simulink model "sst_cllc_dcx_35kHz"  (R2026b)
settings: Solver=ode23tb  StopTime=param.sim.simlength  FixedStep=tc  MaxStep=param.glb_time.tc
values from neighbouring files (symbols this model uses):
  param = struct()    [init_model.m]
libraries: fl_lib x144, nesl_utility x71, mos_simple_2th_lib x8, discrete_time_low_pass_filter x2, lithium_ion_battery x1, single_phase_transformer x1, dab_single_phase_pwm_modulator x1, ee_lib x1
(part 1 of 4)
settings Model: Creator=LTNBDA  LastModifiedBy=d.bagnara
settings SolverCC: AutoInsertRateTranBlk=on  SolverResetMethod=Robust  ZeroCrossAlgorithm=Adaptive  ZeroCrossControl=EnableAll
settings DataIOCC: DSMLogging=off  LimitDataPoints=on  MaxDataPoints=1  ReturnWorkspaceOutputs=off  SaveFormat=Array  SaveOutput=off  SaveTime=off  SignalLogging=off  SignalLoggingSaveFormat=ModelDataLogs
settings OptimizationCC: EfficientMapNaN2IntZero=off  LifeSpan=inf  MemsetInitFltsAndDblsToZero=off
settings DebuggingCC: ArithmeticOperatorsInVariantConditions=warning  FcnCallInpInsideContextMsg=warning  MergeDetectMultiDrivingBlocksExec=none  MultiTaskCondExecSysMsg=none  MultiTaskDSMMsg=warning  MultiTaskRateTransMsg=warning  SFNoUnconditionalDefaultTransitionDiag=warning  SFUnexpectedBacktrackingDiag=warning  SaveWithParameterizedLinksMsg=none  SignalResolutionControl=TryResolveAllWithWarning  SolverPrmCheckMsg=warning  StateNameClashWarn=warning
settings HardwareCC: ProdEndianess=Unspecified  ProdEqTarget=off  ProdHWDeviceType=Generic->64-bit Embedded Processor (LP64)  ProdIntDivRoundTo=Undefined  ProdLargestAtomicFloat=None  TargetEndianess=LittleEndian  TargetHWDeviceType=MATLAB Host  TargetIntDivRoundTo=Zero  TargetLongLongMode=on
settings ModelReferenceCC: PropagateSignalLabelsOutOfModel=off
settings SFSimCC: CustomCodeUndefinedFunction=UseInterfaceOnly  SimUseLocalCustomCode=off
settings SFSimCC: SimCustomHeaderCode=|
  | #include "rpi.h"
  | #include "rpi_simulink.h"
  | #include "mavgflt.h"
  | #include "mavgflt_simulink.h"
  | #include "bemf_obsv.h"
  | #include "bemf_obsv_simulink.h"
  | #include "bemf_obsv_load_est.h"
  | #include "bemf_obsv_load_est_simulink.h"
  | #include "dqvector_pi.h"
  | #include "dqvector_pi_simulink.h"
  | #include "sv_pwm_simulink.h"
  | #include "sv_pwm.h"
  | #include "first_harmonic_tracker.h"
  | #include "first_harmonic_tracker_simulink.h"
  | #include "dqpll_thyr.h"
  | #include "dqpll_thyr_simulink.h"
  | #include "dqpll_grid.h"
  | #include "dqpll_grid_simulink.h"
settings SFSimCC: SimUserIncludeDirs=|
  | include
  | src
settings SFSimCC: SimUserSources=|
  | "mavgflt_simulink.c"
  | "mavgflt.c"
  | "bemf_obsv_simulink.c"
  | "bemf_obsv.c"
  | "bemf_obsv_load_est_simulink.c"
  | "bemf_obsv_load_est.c"
  | "dqvector_pi.c"
  | "dqvector_pi_simulink.c"
  | "sv_pwm_simulink.c"
  | "sv_pwm.c"
  | "first_harmonic_tracker_simulink.c"
  | "first_harmonic_tracker.c"
  | "dqpll_thyr_simulink.c"
  | "dqpll_thyr.c"
  | "dqpll_grid_simulink.c"
  | "dqpll_grid.c"
  | "rpi_simulink.c"
  | "rpi.c"
settings RTWCC: RTWUseLocalCustomCode=off
settings CodeAppCC: StateflowObjectComments=on
settings GRTTargetCC: CombineOutputUpdateFcns=off  GRTInterface=on  TargetLangStandard=C89/C90 (ANSI)
settings ConfigComp: CovExternalEMLEnable=off  CovSaveCumulativeToWorkspaceVar=on  CovSaveSingleToWorkspaceVar=on
settings SimscapeCC: SimscapeNormalizeSystem=off  SimscapeUseEnergyAccounting=off

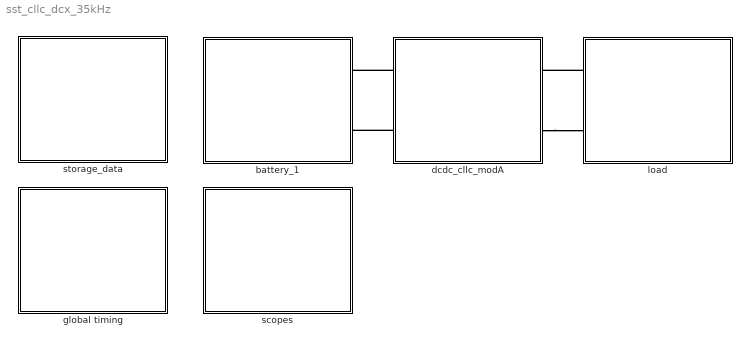
== system sst_cllc_dcx_35kHz ==
  battery_1 : Subsystem
  dcdc_cllc_modA : Subsystem
  global timing : Subsystem
  load : Subsystem
  scopes : Subsystem
  storage_data : Subsystem
  connections:
  dcdc_cllc_modA/LConn1 -- battery_1/RConn1
  dcdc_cllc_modA/LConn2 -- battery_1/RConn2
  load/LConn1 -- dcdc_cllc_modA/RConn1
  dcdc_cllc_modA/RConn2 -- load/LConn2

== system sst_cllc_dcx_35kHz/battery_1 ==
  Electrical Reference1 : fl_lib/Electrical/Electrical Elements/Electrical Reference
  Resistor : fl_lib/Electrical/Electrical Elements/Resistor  Commented=on  R=param.cllc.sink.R1 Ohm  i_specify=off  i_priority=None  i=0 A  i_nominal_specify=off  i_nominal_value=1  i_nominal_unit=A  v_specify=off  v_priority=None  v=0 V  v_nominal_specify=off  v_nominal_value=1  v_nominal_unit=V
  Solver Configuration : nesl_utility/Solver Configuration  PhysicalDomain=network_engine_domain  SubClassName=solver  LeftPortType=input  RightPortType=generic  Tones=[]  Harmonics=[]  SimulateNoise=off  Profile=off  UseLocalSampling=off  EnableSwitchedLinearOptims=on  FrequencyDomain=off  UseCCode=off  RelTol=0.001  AbsTol=0.001  MinStep=1e-09  ToWorkspace=off  RevertToSquareIcSolve=off  NumHomotopyIterations=100  PhasorMode=off  PhasorModeNumHarmonics=1  ConsistencySolver=NEWTON_FTOL  CanonicalOrdering=UNORDERED  OptimizeIntermediates=UNOPTIMIZED  MulticoreSolverChoice=BACKWARD_EULER  IndexReductionMethod=DerivativeReplacement  DoDC=on  ResidualTolerance=1e-5  ConsistencyTolSource=GLOBAL  ConsistencyAbsTol=0.001  ConsistencyRelTol=0.001  ConsistencyTolFactor=0.001  UseLocalSolver=on  LocalSolverChoice=NE_BACKWARD_EULER_ADVANCER  ResolveIndetEquations=on  FunctionEvalNumThread=1  LocalSolverSampleTime=param.glb_time.tc  DoFixedCost=on  MaxNonlinIter=param.sim.nonlinear_iterations  MaxModeIter=2  ComputeImpulses=off  ImpulseIterations=2  LinearAlgebra=auto  LinearAlgebraNumThread=0  EquationFormulation=NE_TIME_EF  DelaysMemoryBudget=1024  AutomaticFiltering=on  FilteringTimeConstant=0.001  PartitionStorageMethod=AS_NEEDED  PartitionMemoryBudget=1024  PartitionMethod=BALANCED  MultibodyUseLocalSolver=off  MultibodyLocalSolverChoice=ODE1  MultibodyLocalSolverSampleTime=0.001
  To Workspace14 : ToWorkspace  VariableName=battery_1_data_sim  SampleTime=param.glb_time.tc
      settings: MaxDataPoints=param.glb_time.Nc  Decimation=param.glb_time.decimation_tc
  lithium ion battery : Scope
      settings: ActiveDisplayYMinimum=-190.26234523392469  ActiveDisplayYMaximum=789.35449820003043  DataLoggingVariableName=ScopeData3
  lithium_ion_battery : lithium_ion_battery/lithium_ion_battery  Q=param.battery.pack_1.Q  number_of_cells=param.battery.pack_1.number_of_cells  E_1=param.battery.pack_1.E_1  E0=param.battery.pack_1.E0  E1=param.battery.pack_1.E1  E2=param.battery.pack_1.E2  E3=param.battery.pack_1.E3  Elog=param.battery.pack_1.Elog  R0=param.battery.pack_1.R0  R1=param.battery.pack_1.R1  C1=param.battery.pack_1.C1  M=param.battery.pack_1.M  alpha=param.battery.pack_1.alpha  soc_init=param.battery.pack_1.soc_init  ts_battery=param.glb_time.ts_dab  q1Kalman=param.battery.pack_1.q1Kalman  q2Kalman=param.battery.pack_1.q2Kalman  q3Kalman=param.battery.pack_1.q3Kalman  rKalman=param.battery.pack_1.rKalman  tc=param.glb_time.tc  enable_white_noise_m=1  battery_voltage_init_m=param.battery.nominal_battery_voltage_1
  single_phase_ui_measure : Subsystem
  dc(+) : PMIOPort  Side=Right
  dc(-) : PMIOPort  Port=2  Side=Right
  wires:
  lithium_ion_battery/1 -> To Workspace14/1, lithium ion battery/1
  connections:
  lithium_ion_battery/RConn2 -- Resistor/RConn1 -- single_phase_ui_measure/LConn2 -- Electrical Reference1/LConn1 -- Solver Configuration/RConn1
  single_phase_ui_measure/RConn1 -- dc(+)/RConn1
  single_phase_ui_measure/LConn1 -- Resistor/LConn1 -- lithium_ion_battery/RConn1
  dc(-)/RConn1 -- single_phase_ui_measure/RConn2

== system sst_cllc_dcx_35kHz/dcdc_cllc_modA ==
  dc/dc with galvanic isolation : Subsystem
  input_current_control : Subsystem
  udc(+) : PMIOPort  Side=Right
  udc(-) : PMIOPort  Port=2  Side=Right
  dc(+) : PMIOPort  Port=3  Side=Left
  dc(-) : PMIOPort  Port=4  Side=Left
  wires:
  input_current_control/1(gate_cmds) -> dc/dc with galvanic isolation/1(dab_gate_cmds)
  connections:
  udc(+)/RConn1 -- dc/dc with galvanic isolation/RConn1
  udc(-)/RConn1 -- dc/dc with galvanic isolation/RConn2
  dc(-)/RConn1 -- dc/dc with galvanic isolation/LConn2
  dc(+)/RConn1 -- dc/dc with galvanic isolation/LConn1

== system sst_cllc_dcx_35kHz/global timing ==
  Unit Delay : UnitDelay  SampleTime=param.glb_time.tc
  time_afe1 : Subsystem  mask{k=1}
      mask prompts: k "Time Gain"
      mask Display:
      | disp('time-gen');
      | port_label('input', 1, 'crt');
      | port_label('output', 1, 'tout');
  time_afe3 : Subsystem  mask{k=1}
      mask prompts: k "Time Gain"
      mask Display:
      | disp('time-gen');
      | port_label('output', 1, 'tout');
  tag scope: time_cllc_module_1=global, time_master=global
  wires:
  time_afe1/1(Out1) -> [time_cllc_module_1]
  time_afe3/1(Out1) -> [time_master]
  [local_time_corr_llc_mod1] -> Unit Delay/1
  Unit Delay/1 -> time_afe1/1(correction_time)

== system sst_cllc_dcx_35kHz/load ==
  Clock : Clock  Commented=on
  Controlled Current Source : fl_lib/Electrical/Electrical Sources/Controlled Current Source  Commented=on
  Electrical Reference1 : fl_lib/Electrical/Electrical Elements/Electrical Reference
  Gain : Gain  Commented=on  Gain=1/param.cllc.sink.t_ramp
  Gain1 : Gain  Commented=on  Gain=param.cllc.sink.I2
  Saturation : Saturate  Commented=on  UpperLimit=1  LowerLimit=0
  Simulink-PS Converter : nesl_utility/Simulink-PS Converter  Commented=on  PhysicalDomain=network_engine_domain  SubClassName=ps_input  LeftPortType=input  RightPortType=output  PseudoPeriodic=off  Frequencies=[]  NoiseDistribution=none  NoiseParameters=[]  Unit=A  AffineConversion=off  FilteringAndDerivatives=provide  SimscapeFilterOrder=1  InputFilterTimeConstant=0.001  UdotUserProvided=0
  Voltage Source : ee_lib/Sources/Voltage Source  Commented=on  dc_voltage=param.cllc.sink.U2 V  ac_voltage=0 V  ac_shift=0 rad  ac_frequency=0 Hz  noise_mode=ee.enum.sources.noise.Disabled  PSD=0 V^2/Hz  sample_time=1e-3 s  repeatability=ee.enum.sources.repeatability.NotRepeatable  user_seed=0  auto_seed=3499211588  i_specify=off  i_priority=None  i=0 A  i_nominal_specify=off  i_nominal_value=1  i_nominal_unit=A  v_specify=off  v_priority=None  v=0 V  v_nominal_specify=off  v_nominal_value=1  v_nominal_unit=V
  passive load : Subsystem
  uload(+) : PMIOPort  Side=Left
  uload(-) : PMIOPort  Port=2  Side=Left
  wires:
  Clock/1 -> Gain/1
  Gain/1 -> Saturation/1
  Saturation/1 -> Gain1/1
  Gain1/1 -> Simulink-PS Converter/1
  connections:
  uload(-)/RConn1 -- Controlled Current Source/LConn1 -- Voltage Source/RConn1 -- Electrical Reference1/LConn1 -- passive load/RConn1
  passive load/LConn1 -- Controlled Current Source/RConn2 -- Voltage Source/LConn1 -- uload(+)/RConn1
  Simulink-PS Converter/RConn1 -- Controlled Current Source/RConn1

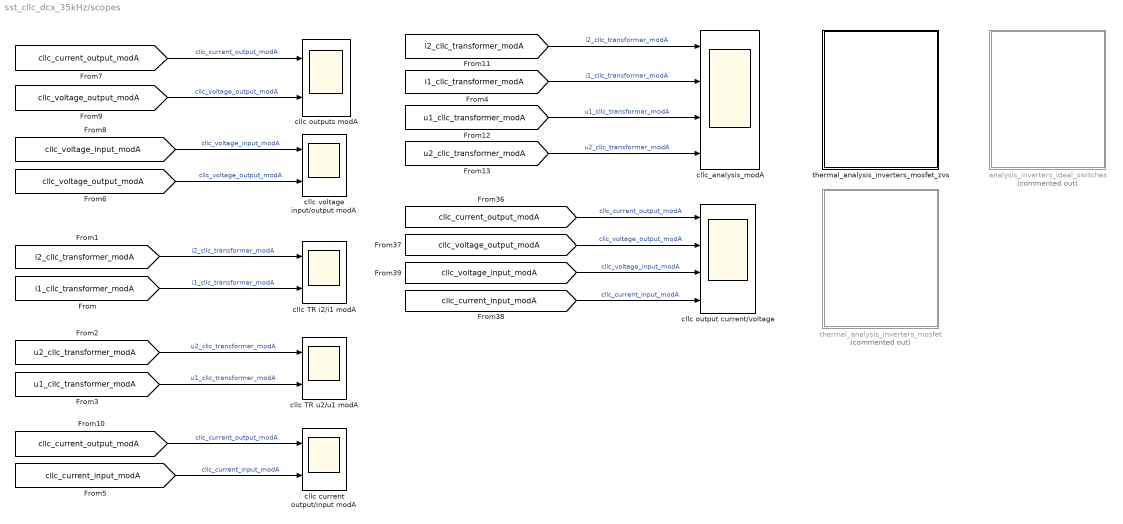
== system sst_cllc_dcx_35kHz/scopes ==
  analysis_inverters_ideal_switches : Subsystem  Commented=on
  cllc TR i2/i1 modA : Scope  NumInputPorts=2
      settings: SampleTime=param.glb_time.tc  ActiveDisplayYMinimum=-621.44843192916471  ActiveDisplayYMaximum=621.071538249071  DataLoggingVariableName=ScopeData13
  cllc TR u2/u1 modA : Scope  NumInputPorts=2
      settings: SampleTime=param.glb_time.tc  ActiveDisplayYMinimum=-1427.1389570347349  ActiveDisplayYMaximum=1427.1405694303187  DataLoggingVariableName=ScopeData4
  cllc current output/input modA : Scope  NumInputPorts=2
      settings: SampleTime=param.glb_time.tc  ActiveDisplayYMinimum=-7.8124999999999982  ActiveDisplayYMaximum=70.3125  DataLoggingVariableName=ScopeData8
  cllc output current/voltage : Scope  NumInputPorts=4
      settings: ActiveDisplayString=3  ActiveDisplayYMinimum=656.54883928896152  ActiveDisplayYMaximum=674.48308776467979  DataLoggingVariableName=ScopeData9
  cllc outputs modA : Scope  NumInputPorts=2
      settings: ActiveDisplayYMinimum=791.98525003287466  ActiveDisplayYMaximum=792.09422024718685  DataLoggingVariableName=ScopeData6
  cllc voltage input/output modA : Scope  NumInputPorts=2
      settings: ActiveDisplayYMinimum=778.88698009854056  ActiveDisplayYMaximum=810.81441530748316  DataLoggingVariableName=ScopeData10
  cllc_analysis_modA : Scope  NumInputPorts=4
      settings: ActiveDisplayYMinimum=-2946.4603447985373  ActiveDisplayYMaximum=3872.2014328676551  DataLoggingVariableName=ScopeData15
  thermal_analysis_inverters_mosfet : Subsystem  Commented=on
  thermal_analysis_inverters_mosfet_zvs : Subsystem
  wires:
  [u2_cllc_transformer_modA] -> cllc TR u2/u1 modA/1  "u2_cllc_transformer_modA"
  [i1_cllc_transformer_modA] -> cllc_analysis_modA/2  "i1_cllc_transformer_modA"
  [cllc_current_output_modA] -> cllc current output/input modA/1  "cllc_current_output_modA"
  [cllc_current_input_modA] -> cllc current output/input modA/2  "cllc_current_input_modA"
  [cllc_voltage_output_modA] -> cllc outputs modA/2  "cllc_voltage_output_modA"
  [cllc_current_output_modA] -> cllc outputs modA/1  "cllc_current_output_modA"
  [i2_cllc_transformer_modA] -> cllc_analysis_modA/1  "i2_cllc_transformer_modA"
  [cllc_voltage_output_modA] -> cllc output current/voltage/2  "cllc_voltage_output_modA"
  [u1_cllc_transformer_modA] -> cllc_analysis_modA/3  "u1_cllc_transformer_modA"
  [cllc_voltage_output_modA] -> cllc voltage input/output modA/2  "cllc_voltage_output_modA"
  [i1_cllc_transformer_modA] -> cllc TR i2/i1 modA/2  "i1_cllc_transformer_modA"
  [cllc_current_input_modA] -> cllc output current/voltage/4  "cllc_current_input_modA"
  [i2_cllc_transformer_modA] -> cllc TR i2/i1 modA/1  "i2_cllc_transformer_modA"
  [cllc_voltage_input_modA] -> cllc voltage input/output modA/1  "cllc_voltage_input_modA"
  [u1_cllc_transformer_modA] -> cllc TR u2/u1 modA/2  "u1_cllc_transformer_modA"
  [u2_cllc_transformer_modA] -> cllc_analysis_modA/4  "u2_cllc_transformer_modA"
  [cllc_voltage_input_modA] -> cllc output current/voltage/3  "cllc_voltage_input_modA"
  [cllc_current_output_modA] -> cllc output current/voltage/1  "cllc_current_output_modA"

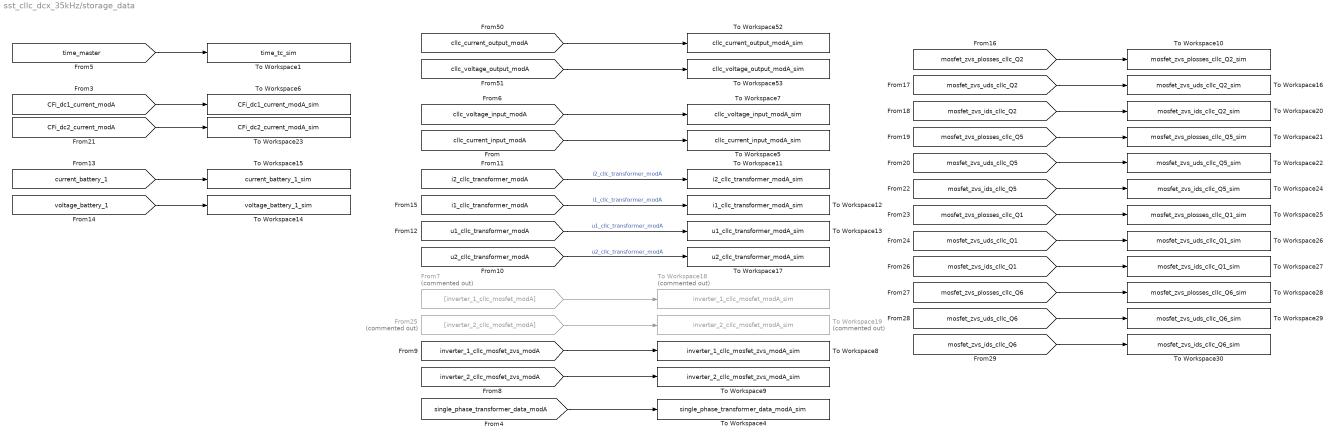
== system sst_cllc_dcx_35kHz/storage_data ==
  From25 : From  Commented=on  GotoTag=inverter_2_cllc_mosfet_modA
  From7 : From  Commented=on  GotoTag=inverter_1_cllc_mosfet_modA
  To Workspace1 : ToWorkspace  VariableName=time_tc_sim  SampleTime=param.glb_time.tc
      settings: MaxDataPoints=param.glb_time.Nc  Decimation=param.glb_time.decimation_tc
  To Workspace10 : ToWorkspace  VariableName=mosfet_zvs_plosses_cllc_Q2_sim  SampleTime=param.glb_time.tc
      settings: MaxDataPoints=param.glb_time.Nc  Decimation=param.glb_time.decimation_tc
  To Workspace11 : ToWorkspace  VariableName=i2_cllc_transformer_modA_sim  SampleTime=param.glb_time.tc
      settings: MaxDataPoints=param.glb_time.Nc  Decimation=param.glb_time.decimation_tc
  To Workspace12 : ToWorkspace  VariableName=i1_cllc_transformer_modA_sim  SampleTime=param.glb_time.tc
      settings: MaxDataPoints=param.glb_time.Nc  Decimation=param.glb_time.decimation_tc
  To Workspace13 : ToWorkspace  VariableName=u1_cllc_transformer_modA_sim  SampleTime=param.glb_time.tc
      settings: MaxDataPoints=param.glb_time.Nc  Decimation=param.glb_time.decimation_tc
  To Workspace14 : ToWorkspace  VariableName=voltage_battery_1_sim  SampleTime=param.glb_time.tc
      settings: MaxDataPoints=param.glb_time.Nc  Decimation=param.glb_time.decimation_tc
  To Workspace15 : ToWorkspace  VariableName=current_battery_1_sim  SampleTime=param.glb_time.tc
      settings: MaxDataPoints=param.glb_time.Nc  Decimation=param.glb_time.decimation_tc
  To Workspace16 : ToWorkspace  VariableName=mosfet_zvs_uds_cllc_Q2_sim  SampleTime=param.glb_time.tc
      settings: MaxDataPoints=param.glb_time.Nc  Decimation=param.glb_time.decimation_tc
  To Workspace17 : ToWorkspace  VariableName=u2_cllc_transformer_modA_sim  SampleTime=param.glb_time.tc
      settings: MaxDataPoints=param.glb_time.Nc  Decimation=param.glb_time.decimation_tc
  To Workspace18 : ToWorkspace  Commented=on  VariableName=inverter_1_cllc_mosfet_modA_sim  SampleTime=param.glb_time.tc
      settings: MaxDataPoints=param.glb_time.Nc  Decimation=param.glb_time.decimation_tc
  To Workspace19 : ToWorkspace  Commented=on  VariableName=inverter_2_cllc_mosfet_modA_sim  SampleTime=param.glb_time.tc
      settings: MaxDataPoints=param.glb_time.Nc  Decimation=param.glb_time.decimation_tc
  To Workspace20 : ToWorkspace  VariableName=mosfet_zvs_ids_cllc_Q2_sim  SampleTime=param.glb_time.tc
      settings: MaxDataPoints=param.glb_time.Nc  Decimation=param.glb_time.decimation_tc
  To Workspace21 : ToWorkspace  VariableName=mosfet_zvs_plosses_cllc_Q5_sim  SampleTime=param.glb_time.tc
      settings: MaxDataPoints=param.glb_time.Nc  Decimation=param.glb_time.decimation_tc
  To Workspace22 : ToWorkspace  VariableName=mosfet_zvs_uds_cllc_Q5_sim  SampleTime=param.glb_time.tc
      settings: MaxDataPoints=param.glb_time.Nc  Decimation=param.glb_time.decimation_tc
  To Workspace23 : ToWorkspace  VariableName=CFi_dc2_current_modA_sim  SampleTime=param.glb_time.tc
      settings: MaxDataPoints=param.glb_time.Nc  Decimation=param.glb_time.decimation_tc
  To Workspace24 : ToWorkspace  VariableName=mosfet_zvs_ids_cllc_Q5_sim  SampleTime=param.glb_time.tc
      settings: MaxDataPoints=param.glb_time.Nc  Decimation=param.glb_time.decimation_tc
  To Workspace25 : ToWorkspace  VariableName=mosfet_zvs_plosses_cllc_Q1_sim  SampleTime=param.glb_time.tc
      settings: MaxDataPoints=param.glb_time.Nc  Decimation=param.glb_time.decimation_tc
  To Workspace26 : ToWorkspace  VariableName=mosfet_zvs_uds_cllc_Q1_sim  SampleTime=param.glb_time.tc
      settings: MaxDataPoints=param.glb_time.Nc  Decimation=param.glb_time.decimation_tc
  To Workspace27 : ToWorkspace  VariableName=mosfet_zvs_ids_cllc_Q1_sim  SampleTime=param.glb_time.tc
      settings: MaxDataPoints=param.glb_time.Nc  Decimation=param.glb_time.decimation_tc
  To Workspace28 : ToWorkspace  VariableName=mosfet_zvs_plosses_cllc_Q6_sim  SampleTime=param.glb_time.tc
      settings: MaxDataPoints=param.glb_time.Nc  Decimation=param.glb_time.decimation_tc
  To Workspace29 : ToWorkspace  VariableName=mosfet_zvs_uds_cllc_Q6_sim  SampleTime=param.glb_time.tc
      settings: MaxDataPoints=param.glb_time.Nc  Decimation=param.glb_time.decimation_tc
  To Workspace30 : ToWorkspace  VariableName=mosfet_zvs_ids_cllc_Q6_sim  SampleTime=param.glb_time.tc
      settings: MaxDataPoints=param.glb_time.Nc  Decimation=param.glb_time.decimation_tc
  To Workspace4 : ToWorkspace  VariableName=single_phase_transformer_data_modA_sim  SampleTime=param.glb_time.tc
      settings: MaxDataPoints=param.glb_time.Nc  Decimation=param.glb_time.decimation_tc
  To Workspace5 : ToWorkspace  VariableName=cllc_current_input_modA_sim  SampleTime=param.glb_time.tc
      settings: MaxDataPoints=param.glb_time.Nc  Decimation=param.glb_time.decimation_tc
  To Workspace52 : ToWorkspace  VariableName=cllc_current_output_modA_sim  SampleTime=param.glb_time.tc
      settings: MaxDataPoints=param.glb_time.Nc  Decimation=param.glb_time.decimation_tc
  To Workspace53 : ToWorkspace  VariableName=cllc_voltage_output_modA_sim  SampleTime=param.glb_time.tc
      settings: MaxDataPoints=param.glb_time.Nc  Decimation=param.glb_time.decimation_tc
  To Workspace6 : ToWorkspace  VariableName=CFi_dc1_current_modA_sim  SampleTime=param.glb_time.tc
      settings: MaxDataPoints=param.glb_time.Nc  Decimation=param.glb_time.decimation_tc
  To Workspace7 : ToWorkspace  VariableName=cllc_voltage_input_modA_sim  SampleTime=param.glb_time.tc
      settings: MaxDataPoints=param.glb_time.Nc  Decimation=param.glb_time.decimation_tc
  To Workspace8 : ToWorkspace  VariableName=inverter_1_cllc_mosfet_zvs_modA_sim  SampleTime=param.glb_time.tc
      settings: MaxDataPoints=param.glb_time.Nc  Decimation=param.glb_time.decimation_tc
  To Workspace9 : ToWorkspace  VariableName=inverter_2_cllc_mosfet_zvs_modA_sim  SampleTime=param.glb_time.tc
      settings: MaxDataPoints=param.glb_time.Nc  Decimation=param.glb_time.decimation_tc
  wires:
  [CFi_dc1_current_modA] -> To Workspace6/1
  [cllc_voltage_input_modA] -> To Workspace7/1
  [voltage_battery_1] -> To Workspace14/1
  [current_battery_1] -> To Workspace15/1
  [CFi_dc2_current_modA] -> To Workspace23/1
  [cllc_voltage_output_modA] -> To Workspace53/1
  [cllc_current_output_modA] -> To Workspace52/1
  [cllc_current_input_modA] -> To Workspace5/1
  [i2_cllc_transformer_modA] -> To Workspace11/1  "i2_cllc_transformer_modA"
  [i1_cllc_transformer_modA] -> To Workspace12/1  "i1_cllc_transformer_modA"
  [u1_cllc_transformer_modA] -> To Workspace13/1  "u1_cllc_transformer_modA"
  [u2_cllc_transformer_modA] -> To Workspace17/1  "u2_cllc_transformer_modA"
  From7/1 -> To Workspace18/1
  From25/1 -> To Workspace19/1
  [single_phase_transformer_data_modA] -> To Workspace4/1
  [time_master] -> To Workspace1/1
  [inverter_2_cllc_mosfet_zvs_modA] -> To Workspace9/1
  [inverter_1_cllc_mosfet_zvs_modA] -> To Workspace8/1
  [mosfet_zvs_plosses_cllc_Q2] -> To Workspace10/1
  [mosfet_zvs_uds_cllc_Q2] -> To Workspace16/1
  [mosfet_zvs_ids_cllc_Q2] -> To Workspace20/1
  [mosfet_zvs_uds_cllc_Q5] -> To Workspace22/1
  [mosfet_zvs_plosses_cllc_Q5] -> To Workspace21/1
  [mosfet_zvs_ids_cllc_Q5] -> To Workspace24/1
  [mosfet_zvs_ids_cllc_Q6] -> To Workspace30/1
  [mosfet_zvs_plosses_cllc_Q6] -> To Workspace28/1
  [mosfet_zvs_uds_cllc_Q6] -> To Workspace29/1
  [mosfet_zvs_ids_cllc_Q1] -> To Workspace27/1
  [mosfet_zvs_uds_cllc_Q1] -> To Workspace26/1
  [mosfet_zvs_plosses_cllc_Q1] -> To Workspace25/1

== system sst_cllc_dcx_35kHz/battery_1/single_phase_ui_measure ==
  Bus Creator : BusCreator  Inputs=2
  Current Sensor : fl_lib/Electrical/Electrical Sensors/Current Sensor
  Selector : Selector  InputPortWidth=2  IndexOptions=Index vector (dialog)  Indices=2  OutputSizes=1  RuntimeRangeChecks=off
  Selector1 : Selector  InputPortWidth=2  IndexOptions=Index vector (dialog)  Indices=1  OutputSizes=1  RuntimeRangeChecks=off
  Voltage Sensor : fl_lib/Electrical/Electrical Sensors/Voltage Sensor
  dab input modA : Scope  NumInputPorts=2
      settings: SampleTime=param.glb_time.tc  ActiveDisplayYMinimum=-99.874352858811619  ActiveDisplayYMaximum=11.097301481144559  DataLoggingVariableName=ScopeData2
  iph : nesl_utility/PS-Simulink Converter  PhysicalDomain=network_engine_domain  SubClassName=ps_output  LeftPortType=input  RightPortType=output  PseudoPeriodic=off  Frequencies=[]  VectorFormat=1-D array  Unit=A  AffineConversion=off
  uph : nesl_utility/PS-Simulink Converter  PhysicalDomain=network_engine_domain  SubClassName=ps_output  LeftPortType=input  RightPortType=output  PseudoPeriodic=off  Frequencies=[]  VectorFormat=1-D array  Unit=V  AffineConversion=off
  Udc(+) : PMIOPort  Side=Left
  udc(+) : PMIOPort  Port=2  Side=Right
  Udc(-) : PMIOPort  Port=3  Side=Left
  udc(-) : PMIOPort  Port=4  Side=Right
  tag scope: current_battery_1=global, voltage_battery_1=global
  wires:
  Bus Creator/1 -> Selector/1, Selector1/1  "ui_data"
  iph/1 -> Bus Creator/1  "iph"
  uph/1 -> Bus Creator/2  "uph"
  Selector1/1 -> [current_battery_1], dab input modA/1  "current_battery"
  Selector/1 -> dab input modA/2, [voltage_battery_1]  "voltage_battery"
  connections:
  iph/LConn1 -- Current Sensor/RConn1
  Voltage Sensor/LConn1 -- Current Sensor/LConn1 -- Udc(+)/RConn1
  Current Sensor/RConn2 -- udc(+)/RConn1
  Voltage Sensor/RConn1 -- uph/LConn1
  Voltage Sensor/RConn2 -- Udc(-)/RConn1 -- udc(-)/RConn1

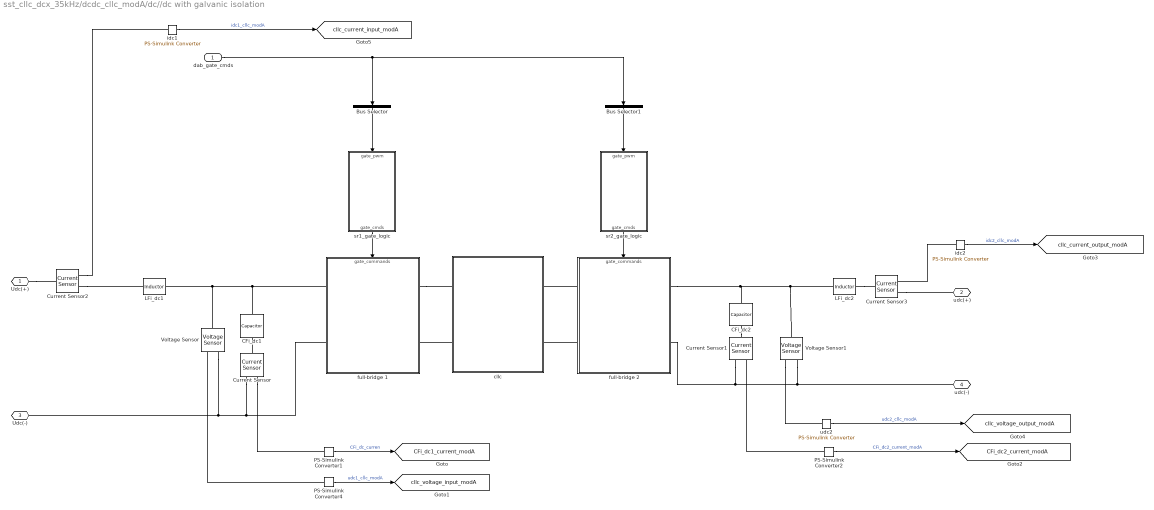
== system sst_cllc_dcx_35kHz/dcdc_cllc_modA/dc//dc with galvanic isolation ==
  dab_gate_cmds : Inport
  Bus Selector : BusSelector  OutputSignals=full_bridge1.gate_cmd_Q1,full_bridge1.gate_cmd_Q2,full_bridge1.gate_cmd_Q3,full_bridge1.gate_cmd_Q4  OutputAsBus=on
  Bus Selector1 : BusSelector  OutputSignals=full_bridge2.gate_cmd_Q1,full_bridge2.gate_cmd_Q2,full_bridge2.gate_cmd_Q3,full_bridge2.gate_cmd_Q4  OutputAsBus=on
  CFi_dc1 : fl_lib/Electrical/Electrical Elements/Capacitor  c=param.cllc.hw.Cdc_dc1 F  r=param.cllc.hw.RCdc_dc1 Ohm  g=0 1/Ohm  i_specify=off  i_priority=None  i=0 A  i_nominal_specify=off  i_nominal_value=1  i_nominal_unit=A  v_specify=on  v_priority=High  v=param.cllc.ic.vc_dc1 V  v_nominal_specify=off  v_nominal_value=1  v_nominal_unit=V  vc_specify=off  vc_priority=High  vc=0 V  vc_nominal_specify=off  vc_nominal_value=1  vc_nominal_unit=V
  CFi_dc2 : fl_lib/Electrical/Electrical Elements/Capacitor  c=param.cllc.hw.Cdc_dc2 F  r=param.cllc.hw.RCdc_dc2 Ohm  g=0 1/Ohm  i_specify=off  i_priority=None  i=0 A  i_nominal_specify=off  i_nominal_value=1  i_nominal_unit=A  v_specify=on  v_priority=High  v=param.cllc.ic.vc_dc2 V  v_nominal_specify=off  v_nominal_value=1  v_nominal_unit=V  vc_specify=off  vc_priority=High  vc=0 V  vc_nominal_specify=off  vc_nominal_value=1  vc_nominal_unit=V
  Current Sensor{,1..3} (4 alike) : fl_lib/Electrical/Electrical Sensors/Current Sensor
  LFi_dc1 : fl_lib/Electrical/Electrical Elements/Inductor  l=param.cllc.hw.Ldc_dc1 H  r=param.cllc.hw.RLdc_dc1 Ohm  g=1e-9 1/Ohm  i_specify=off  i_priority=None  i=0 A  i_nominal_specify=off  i_nominal_value=1  i_nominal_unit=A  v_specify=off  v_priority=None  v=0 V  v_nominal_specify=off  v_nominal_value=1  v_nominal_unit=V  i_L_specify=off  i_L_priority=High  i_L=0 A  i_L_nominal_specify=off  i_L_nominal_value=1  i_L_nominal_unit=A
  LFi_dc2 : fl_lib/Electrical/Electrical Elements/Inductor  l=param.cllc.hw.Ldc_dc2 H  r=param.cllc.hw.RLdc_dc2 Ohm  g=1e-9 1/Ohm  i_specify=off  i_priority=None  i=0 A  i_nominal_specify=off  i_nominal_value=1  i_nominal_unit=A  v_specify=off  v_priority=None  v=0 V  v_nominal_specify=off  v_nominal_value=1  v_nominal_unit=V  i_L_specify=off  i_L_priority=High  i_L=0 A  i_L_nominal_specify=off  i_L_nominal_value=1  i_L_nominal_unit=A
  PS-Simulink Converter1 : nesl_utility/PS-Simulink Converter  PhysicalDomain=network_engine_domain  SubClassName=ps_output  LeftPortType=input  RightPortType=output  PseudoPeriodic=off  Frequencies=[]  VectorFormat=1-D array  Unit=A  AffineConversion=on
  PS-Simulink Converter2 : nesl_utility/PS-Simulink Converter  PhysicalDomain=network_engine_domain  SubClassName=ps_output  LeftPortType=input  RightPortType=output  PseudoPeriodic=off  Frequencies=[]  VectorFormat=1-D array  Unit=A  AffineConversion=on
  PS-Simulink Converter4 : nesl_utility/PS-Simulink Converter  PhysicalDomain=network_engine_domain  SubClassName=ps_output  LeftPortType=input  RightPortType=output  PseudoPeriodic=off  Frequencies=[]  VectorFormat=1-D array  Unit=V  AffineConversion=on
  Voltage Sensor : fl_lib/Electrical/Electrical Sensors/Voltage Sensor
  Voltage Sensor1 : fl_lib/Electrical/Electrical Sensors/Voltage Sensor
  cllc : Subsystem
  full-bridge 1 : Subsystem
      settings: PortSchema="{\"entries\":[{\"content\":{\"sides\":[{\"content\":{\"connectorIds\":[\"LConn1\",\"LConn2\"]},\"type\":\"ConnectorPlacement.EquallySpacedRectSide\",\"uuid\":\"c872503a-61af-4937-bdf2-4de4f8645573\"},{\"content\":{\"connectorIds\":[\"RConn1\",\"RConn2\"],\"side\":\"RIGHT\"},\"type\":\"ConnectorPlacement.EquallySpacedRectSide\",\"uuid\":\"3b83f060-86a2-4569-84b5-d9f7c0485347\"},{\"content\":{\"connectorIds\":[\"In1\"],\"side\":\"TOP\"},\"type\":\"ConnectorPlacement.EquallySpacedRectSide\",\"uuid\":\"bf191d46-ce71-4d15-9dd0-24cc57253577\"}]},\"type\":\"ConnectorPlacement.EquallySpacedConnector\",\"uuid\":\"1b28ceee-25d0-45ae-a3c4-c2563f0d63ba\"}],\"packageUris\":[\"http://schema.mathworks.com/mf0/Connector/R2020b\"],\"version\":\"1.0\"}"
  full-bridge 2 : Subsystem
      settings: PortSchema="{\"entries\":[{\"content\":{\"sides\":[{\"content\":{\"connectorIds\":[\"LConn1\",\"LConn2\"]},\"type\":\"ConnectorPlacement.EquallySpacedRectSide\",\"uuid\":\"c872503a-61af-4937-bdf2-4de4f8645573\"},{\"content\":{\"connectorIds\":[\"RConn1\",\"RConn2\"],\"side\":\"RIGHT\"},\"type\":\"ConnectorPlacement.EquallySpacedRectSide\",\"uuid\":\"3b83f060-86a2-4569-84b5-d9f7c0485347\"},{\"content\":{\"connectorIds\":[\"In1\"],\"side\":\"TOP\"},\"type\":\"ConnectorPlacement.EquallySpacedRectSide\",\"uuid\":\"bf191d46-ce71-4d15-9dd0-24cc57253577\"}]},\"type\":\"ConnectorPlacement.EquallySpacedConnector\",\"uuid\":\"1b28ceee-25d0-45ae-a3c4-c2563f0d63ba\"}],\"packageUris\":[\"http://schema.mathworks.com/mf0/Connector/R2020b\"],\"version\":\"1.0\"}"
  idc1 : nesl_utility/PS-Simulink Converter  PhysicalDomain=network_engine_domain  SubClassName=ps_output  LeftPortType=input  RightPortType=output  PseudoPeriodic=off  Frequencies=[]  VectorFormat=1-D array  Unit=A  AffineConversion=on
  idc2 : nesl_utility/PS-Simulink Converter  PhysicalDomain=network_engine_domain  SubClassName=ps_output  LeftPortType=input  RightPortType=output  PseudoPeriodic=off  Frequencies=[]  VectorFormat=1-D array  Unit=A  AffineConversion=off
  sr1_gate_logic : Subsystem
  sr2_gate_logic : Subsystem
  udc2 : nesl_utility/PS-Simulink Converter  PhysicalDomain=network_engine_domain  SubClassName=ps_output  LeftPortType=input  RightPortType=output  PseudoPeriodic=off  Frequencies=[]  VectorFormat=1-D array  Unit=V  AffineConversion=off
  Udc(+) : PMIOPort  Side=Left
  udc(+) : PMIOPort  Port=2  Side=Right
  Udc(-) : PMIOPort  Port=3  Side=Left
  udc(-) : PMIOPort  Port=4  Side=Right
  tag scope: CFi_dc1_current_modA=global, CFi_dc2_current_modA=global, cllc_current_input_modA=global, cllc_current_output_modA=global, cllc_voltage_input_modA=global, cllc_voltage_output_modA=global
  wires:
  PS-Simulink Converter1/1 -> [CFi_dc1_current_modA]  "CFi_dc_curren"
  PS-Simulink Converter4/1 -> [cllc_voltage_input_modA]  "udc1_cllc_modA"
  idc1/1 -> [cllc_current_input_modA]  "idc1_cllc_modA"
  dab_gate_cmds/1 -> Bus Selector/1, Bus Selector1/1
  PS-Simulink Converter2/1 -> [CFi_dc2_current_modA]  "CFi_dc2_current_modA"
  udc2/1 -> [cllc_voltage_output_modA]  "udc2_cllc_modA"
  idc2/1 -> [cllc_current_output_modA]  "idc2_cllc_modA"
  Bus Selector1/1 -> sr2_gate_logic/1(gate_pwm)
  sr2_gate_logic/1(gate_cmds) -> full-bridge 2/1(gate_commands)
  Bus Selector/1 -> sr1_gate_logic/1(gate_pwm)
  sr1_gate_logic/1(gate_cmds) -> full-bridge 1/1(gate_commands)
  connections:
  cllc/LConn2 -- full-bridge 1/LConn2
  full-bridge 1/RConn1 -- CFi_dc1/LConn1 -- Voltage Sensor/LConn1 -- LFi_dc1/RConn1
  Current Sensor/LConn1 -- CFi_dc1/RConn1
  Current Sensor/RConn1 -- PS-Simulink Converter1/LConn1
  PS-Simulink Converter4/LConn1 -- Voltage Sensor/RConn1
  full-bridge 1/LConn1 -- cllc/LConn1
  Current Sensor2/RConn2 -- LFi_dc1/LConn1
  Udc(+)/RConn1 -- Current Sensor2/LConn1
  Current Sensor2/RConn1 -- idc1/LConn1
  full-bridge 2/LConn1 -- cllc/RConn1
  full-bridge 2/LConn2 -- cllc/RConn2
  CFi_dc2/RConn1 -- Current Sensor1/LConn1
  PS-Simulink Converter2/LConn1 -- Current Sensor1/RConn1
  LFi_dc2/LConn1 -- Voltage Sensor1/LConn1 -- full-bridge 2/RConn1 -- CFi_dc2/LConn1
  LFi_dc2/RConn1 -- Current Sensor3/LConn1
  Current Sensor3/RConn2 -- udc(+)/RConn1
  idc2/LConn1 -- Current Sensor3/RConn1
  Voltage Sensor1/RConn1 -- udc2/LConn1
  full-bridge 1/RConn2 -- Current Sensor/RConn2 -- Udc(-)/RConn1 -- Voltage Sensor/RConn2
  Current Sensor1/RConn2 -- full-bridge 2/RConn2 -- udc(-)/RConn1 -- Voltage Sensor1/RConn2

== system sst_cllc_dcx_35kHz/dcdc_cllc_modA/input_current_control ==
  input_current_control : Subsystem  Commented=on
  modulator : Subsystem
  normalization : Subsystem
  gate_cmds : Outport
  wires:
  [cllc_current_input_modA] -> normalization/1(in)
  normalization/1(out_pu) -> input_current_control/1(current_input_pu)
  [TRGO] -> input_current_control/Trigger
  [time_cllc_module_1] -> input_current_control/2(local_time)
  input_current_control/1(ictrl_out) -> modulator/1(phase_displacement)
  modulator/1(gate_cmds) -> gate_cmds/1

== system sst_cllc_dcx_35kHz/global timing/time_afe1 ==
  correction_time : Inport
  Constant : Constant
  Gain : Gain  Gain=k
  Product : Product
  Sum : Sum  Inputs=|++
  time_1 : Clock
  Out1 : Outport
  wires:
  time_1/1 -> Gain/1
  Gain/1 -> Product/1
  Product/1 -> Out1/1
  correction_time/1 -> Sum/1
  Sum/1 -> Product/2
  Constant/1 -> Sum/2

== system sst_cllc_dcx_35kHz/global timing/time_afe3 ==
  Gain : Gain  Gain=k
  time_1 : Clock
  Out1 : Outport
  wires:
  Gain/1 -> Out1/1
  time_1/1 -> Gain/1

== system sst_cllc_dcx_35kHz/load/passive load ==
  load : fl_lib/Electrical/Electrical Elements/Resistor  R=800^2/50e3 Ohm  i_specify=off  i_priority=None  i=0 A  i_nominal_specify=off  i_nominal_value=1  i_nominal_unit=A  v_specify=off  v_priority=None  v=0 V  v_nominal_specify=off  v_nominal_value=1  v_nominal_unit=V
  load(+) : PMIOPort  Side=Left
  load(-) : PMIOPort  Port=2  Side=Right
  connections:
  load(-)/RConn1 -- load/RConn1
  load/LConn1 -- load(+)/RConn1

== system sst_cllc_dcx_35kHz/scopes/analysis_inverters_ideal_switches ==
  cllc_full_bridge_1_analysis : Scope  NumInputPorts=4
      settings: SampleTime=param.glb_time.tc  ActiveDisplayYMinimum=-938.27755511768964  ActiveDisplayYMaximum=1590.9851774094091  DataLoggingVariableName=ScopeData16
  cllc_full_bridge_2_analysis : Scope  NumInputPorts=4
      settings: SampleTime=param.glb_time.tc  ActiveDisplayYMinimum=-41114.10349340782  ActiveDisplayYMaximum=4578.90466536263  DataLoggingVariableName=ScopeData17
  wires:
  [idevice_ids_cllc_Q5] -> cllc_full_bridge_2_analysis/1  "idevice_ids_cllc_Q5"
  [idevice_uds_cllc_Q5] -> cllc_full_bridge_2_analysis/2  "idevice_uds_cllc_Q5"
  [idevice_ids_cllc_Q6] -> cllc_full_bridge_2_analysis/3  "idevice_ids_cllc_Q6"
  [idevice_uds_cllc_Q6] -> cllc_full_bridge_2_analysis/4  "idevice_uds_cllc_Q6"
  [idevice_uds_cllc_Q2] -> cllc_full_bridge_1_analysis/4  "idevice_uds_cllc_Q2"
  [idevice_ids_cllc_Q2] -> cllc_full_bridge_1_analysis/3  "idevice_ids_cllc_Q2"
  [idevice_uds_cllc_Q1] -> cllc_full_bridge_1_analysis/2  "idevice_uds_cllc_Q1"
  [idevice_ids_cllc_Q1] -> cllc_full_bridge_1_analysis/1  "idevice_ids_cllc_Q1"

== system sst_cllc_dcx_35kHz/scopes/thermal_analysis_inverters_mosfet ==
  Bus Selector : BusSelector  OutputSignals=mosfet_ploss_Q1,mosfet_ploss_Q2
  Bus Selector1 : BusSelector  OutputSignals=mosfet_ploss_Q1,mosfet_ploss_Q2
  Bus Selector2 : BusSelector  OutputSignals=mosfet_voltage_Q1,mosfet_voltage_Q2
  Bus Selector4 : BusSelector  OutputSignals=mosfet_current_Q1,mosfet_current_Q2
  Bus Selector5 : BusSelector  OutputSignals=mosfet_voltage_Q1,mosfet_voltage_Q2
  Bus Selector6 : BusSelector  OutputSignals=mosfet_current_Q1,mosfet_current_Q2
  cllc_analysis_full_bridge_1 : Scope  NumInputPorts=4
      settings: SampleTime=param.glb_time.tc  ActiveDisplayYMinimum=-144.60893370238608  ActiveDisplayYMaximum=1256.4324923995921  DataLoggingVariableName=ScopeData5
  cllc_analysis_full_bridge_2 : Scope  NumInputPorts=4
      settings: SampleTime=param.glb_time.tc  ActiveDisplayYMinimum=-2201.7502200164981  ActiveDisplayYMaximum=17169.939546487192  DataLoggingVariableName=ScopeData7
  cllc_analysis_power loss : Scope  NumInputPorts=4
      settings: SampleTime=param.glb_time.tc  ActiveDisplayYMinimum=-12.986178564788585  ActiveDisplayYMaximum=150.90789550701129
  wires:
  Bus Selector1/1 -> cllc_analysis_power loss/3  "<mosfet_ploss_Q1>"
  [inverter_1_cllc_mosfet_modA] -> Bus Selector/1
  Bus Selector1/2 -> cllc_analysis_power loss/4  "<mosfet_ploss_Q2>"
  [inverter_2_cllc_mosfet_modA] -> Bus Selector1/1
  Bus Selector/1 -> cllc_analysis_power loss/1  "<mosfet_ploss_Q1>"
  Bus Selector/2 -> cllc_analysis_power loss/2  "<mosfet_ploss_Q2>"
  [inverter_2_cllc_mosfet_modA] -> Bus Selector6/1, Bus Selector5/1
  [inverter_1_cllc_mosfet_modA] -> Bus Selector4/1, Bus Selector2/1
  Bus Selector2/1 -> cllc_analysis_full_bridge_1/1  "<mosfet_voltage_Q1>"
  Bus Selector2/2 -> cllc_analysis_full_bridge_1/2  "<mosfet_voltage_Q2>"
  Bus Selector4/1 -> cllc_analysis_full_bridge_1/3  "<mosfet_current_Q1>"
  Bus Selector4/2 -> cllc_analysis_full_bridge_1/4  "<mosfet_current_Q2>"
  Bus Selector6/2 -> cllc_analysis_full_bridge_2/4  "<mosfet_current_Q2>"
  Bus Selector6/1 -> cllc_analysis_full_bridge_2/3  "<mosfet_current_Q1>"
  Bus Selector5/2 -> cllc_analysis_full_bridge_2/2  "<mosfet_voltage_Q2>"
  Bus Selector5/1 -> cllc_analysis_full_bridge_2/1  "<mosfet_voltage_Q1>"

== system sst_cllc_dcx_35kHz/scopes/thermal_analysis_inverters_mosfet_zvs ==
  Bus Selector : BusSelector  OutputSignals=mosfet_ploss_Q1,mosfet_ploss_Q2
  Bus Selector1 : BusSelector  OutputSignals=mosfet_ploss_Q1,mosfet_ploss_Q2
  Bus Selector2 : BusSelector  OutputSignals=mosfet_voltage_Q1,mosfet_voltage_Q2
  Bus Selector4 : BusSelector  OutputSignals=mosfet_current_Q1,mosfet_current_Q2
  Bus Selector5 : BusSelector  OutputSignals=mosfet_voltage_Q1,mosfet_voltage_Q2
  Bus Selector6 : BusSelector  OutputSignals=mosfet_current_Q1,mosfet_current_Q2
  cllc_analysis_full_bridge_1 : Scope  NumInputPorts=4
      settings: SampleTime=param.glb_time.tc  ActiveDisplayYMinimum=-147.14952093736252  ActiveDisplayYMaximum=1282.2602375044905  DataLoggingVariableName=ScopeData11
  cllc_analysis_full_bridge_2 : Scope  NumInputPorts=4
      settings: SampleTime=param.glb_time.tc  ActiveDisplayYMinimum=-147.66926705552075  ActiveDisplayYMaximum=1287.1646023554745  DataLoggingVariableName=ScopeData18
  cllc_analysis_power loss : Scope  NumInputPorts=4
      settings: SampleTime=param.glb_time.tc  ActiveDisplayYMinimum=-3.3519856795671767  ActiveDisplayYMaximum=64.171504680220778  DataLoggingVariableName=ScopeData17
  wires:
  Bus Selector1/2 -> cllc_analysis_power loss/4  "<mosfet_ploss_Q2>"
  [inverter_2_cllc_mosfet_zvs_modA] -> Bus Selector1/1
  Bus Selector/1 -> cllc_analysis_power loss/1  "<mosfet_ploss_Q1>"
  Bus Selector/2 -> cllc_analysis_power loss/2  "<mosfet_ploss_Q2>"
  [inverter_1_cllc_mosfet_zvs_modA] -> Bus Selector/1
  Bus Selector1/1 -> cllc_analysis_power loss/3  "<mosfet_ploss_Q1>"
  [inverter_2_cllc_mosfet_zvs_modA] -> Bus Selector6/1, Bus Selector5/1
  Bus Selector5/1 -> cllc_analysis_full_bridge_2/1  "<mosfet_voltage_Q1>"
  Bus Selector5/2 -> cllc_analysis_full_bridge_2/2  "<mosfet_voltage_Q2>"
  Bus Selector6/2 -> cllc_analysis_full_bridge_2/4  "<mosfet_current_Q2>"
  Bus Selector4/2 -> cllc_analysis_full_bridge_1/4  "<mosfet_current_Q2>"
  [inverter_1_cllc_mosfet_zvs_modA] -> Bus Selector4/1, Bus Selector2/1
  Bus Selector2/1 -> cllc_analysis_full_bridge_1/1  "<mosfet_voltage_Q1>"
  Bus Selector6/1 -> cllc_analysis_full_bridge_2/3  "<mosfet_current_Q1>"
  Bus Selector2/2 -> cllc_analysis_full_bridge_1/2  "<mosfet_voltage_Q2>"
  Bus Selector4/1 -> cllc_analysis_full_bridge_1/3  "<mosfet_current_Q1>"

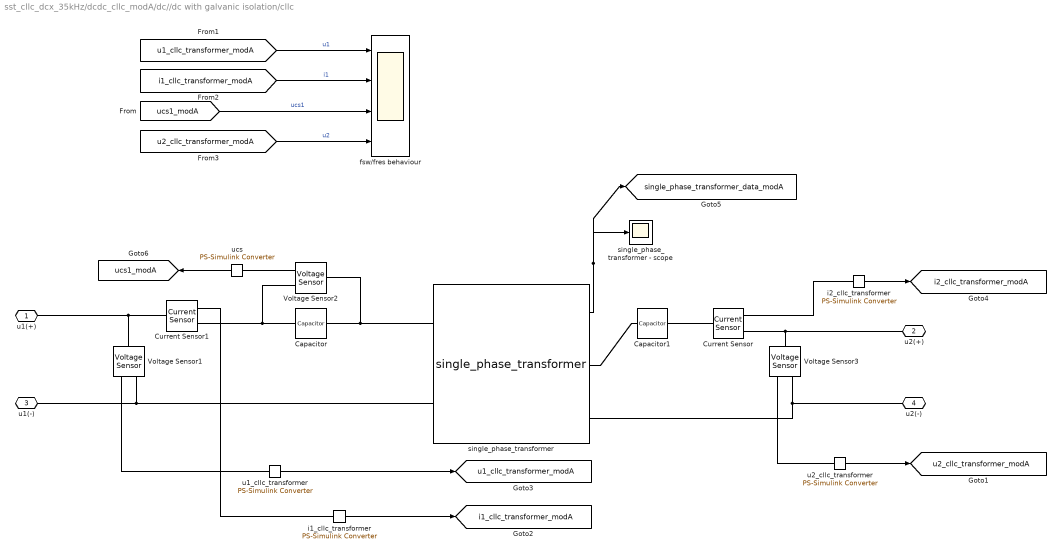
== system sst_cllc_dcx_35kHz/dcdc_cllc_modA/dc//dc with galvanic isolation/cllc ==
  Capacitor : fl_lib/Electrical/Electrical Elements/Capacitor  c=param.cllc.hw.Cs1 F  r=1e-6 Ohm  g=0 1/Ohm  i_specify=off  i_priority=None  i=0 A  i_nominal_specify=off  i_nominal_value=1  i_nominal_unit=A  v_specify=off  v_priority=None  v=0 V  v_nominal_specify=off  v_nominal_value=1  v_nominal_unit=V  vc_specify=off  vc_priority=High  vc=0 V  vc_nominal_specify=off  vc_nominal_value=1  vc_nominal_unit=V
  Capacitor1 : fl_lib/Electrical/Electrical Elements/Capacitor  c=param.cllc.hw.Cs2 F  r=1e-6 Ohm  g=0 1/Ohm  i_specify=off  i_priority=None  i=0 A  i_nominal_specify=off  i_nominal_value=1  i_nominal_unit=A  v_specify=off  v_priority=None  v=0 V  v_nominal_specify=off  v_nominal_value=1  v_nominal_unit=V  vc_specify=off  vc_priority=High  vc=0 V  vc_nominal_specify=off  vc_nominal_value=1  vc_nominal_unit=V
  Current Sensor : fl_lib/Electrical/Electrical Sensors/Current Sensor
  Current Sensor1 : fl_lib/Electrical/Electrical Sensors/Current Sensor
  Voltage Sensor1 : fl_lib/Electrical/Electrical Sensors/Voltage Sensor
  Voltage Sensor2 : fl_lib/Electrical/Electrical Sensors/Voltage Sensor
  Voltage Sensor3 : fl_lib/Electrical/Electrical Sensors/Voltage Sensor
  fsw/fres behaviour : Scope  NumInputPorts=4
      settings: ActiveDisplayYMinimum=-11755.61785973812  ActiveDisplayYMaximum=60393.229814704748  DataLoggingVariableName=ScopeData14
  i1_cllc_transformer : nesl_utility/PS-Simulink Converter  PhysicalDomain=network_engine_domain  SubClassName=ps_output  LeftPortType=input  RightPortType=output  PseudoPeriodic=off  Frequencies=[]  VectorFormat=1-D array  Unit=A  AffineConversion=off
  i2_cllc_transformer : nesl_utility/PS-Simulink Converter  PhysicalDomain=network_engine_domain  SubClassName=ps_output  LeftPortType=input  RightPortType=output  PseudoPeriodic=off  Frequencies=[]  VectorFormat=1-D array  Unit=A  AffineConversion=off
  single_phase_transformer : single_phase_transformer/single_phase_transformer  lm_trafo=param.cllc.hw.Lm  m1=param.cllc.hw.n1  m2=param.cllc.hw.n2  rd1_trafo=param.cllc.hw.Rs1  rd2_trafo=param.cllc.hw.Rs2  ld1_trafo=param.cllc.hw.Ld1  ld2_trafo=param.cllc.hw.Ld2  rfe_trafo=param.cllc.hw.Rfe  length_core=param.cllc.hw.core_length  mu0=1.256637e-6  mur=param.cllc.hw.core_mur
  single_phase_transformer - scope : Scope
      settings: ActiveDisplayYMinimum=-27.208955965522478  ActiveDisplayYMaximum=38.906990847252018  DataLoggingVariableName=ScopeData21
  u1_cllc_transformer : nesl_utility/PS-Simulink Converter  PhysicalDomain=network_engine_domain  SubClassName=ps_output  LeftPortType=input  RightPortType=output  PseudoPeriodic=off  Frequencies=[]  VectorFormat=1-D array  Unit=V  AffineConversion=on
  u2_cllc_transformer : nesl_utility/PS-Simulink Converter  PhysicalDomain=network_engine_domain  SubClassName=ps_output  LeftPortType=input  RightPortType=output  PseudoPeriodic=off  Frequencies=[]  VectorFormat=1-D array  Unit=V  AffineConversion=on
  ucs : nesl_utility/PS-Simulink Converter  PhysicalDomain=network_engine_domain  SubClassName=ps_output  LeftPortType=input  RightPortType=output  PseudoPeriodic=off  Frequencies=[]  VectorFormat=1-D array  Unit=V  AffineConversion=on
  u1(+) : PMIOPort  Side=Left
  u2(+) : PMIOPort  Port=2  Side=Right
  u1(-) : PMIOPort  Port=3  Side=Left
  u2(-) : PMIOPort  Port=4  Side=Right
  tag scope: i1_cllc_transformer_modA=global, i2_cllc_transformer_modA=global, single_phase_transformer_data_modA=global, u1_cllc_transformer_modA=global, u2_cllc_transformer_modA=global, ucs1_modA=global
  wires:
  i2_cllc_transformer/1 -> [i2_cllc_transformer_modA]
  u2_cllc_transformer/1 -> [u2_cllc_transformer_modA]
  u1_cllc_transformer/1 -> [u1_cllc_transformer_modA]
  i1_cllc_transformer/1 -> [i1_cllc_transformer_modA]
  single_phase_transformer/1 -> [single_phase_transformer_data_modA], single_phase_transformer - scope/1
  ucs/1 -> [ucs1_modA]
  [u1_cllc_transformer_modA] -> fsw/fres behaviour/1  "u1"
  [i1_cllc_transformer_modA] -> fsw/fres behaviour/2  "i1"
  [ucs1_modA] -> fsw/fres behaviour/3  "ucs1"
  [u2_cllc_transformer_modA] -> fsw/fres behaviour/4  "u2"
  connections:
  Current Sensor/RConn2 -- Voltage Sensor3/LConn1 -- u2(+)/RConn1
  Voltage Sensor3/RConn2 -- single_phase_transformer/RConn2 -- u2(-)/RConn1
  Current Sensor/RConn1 -- i2_cllc_transformer/LConn1
  Voltage Sensor3/RConn1 -- u2_cllc_transformer/LConn1
  u1(-)/RConn1 -- single_phase_transformer/LConn2 -- Voltage Sensor1/RConn2
  Current Sensor1/LConn1 -- Voltage Sensor1/LConn1 -- u1(+)/RConn1
  Voltage Sensor1/RConn1 -- u1_cllc_transformer/LConn1
  Current Sensor1/RConn1 -- i1_cllc_transformer/LConn1
  Current Sensor/LConn1 -- Capacitor1/RConn1
  single_phase_transformer/LConn1 -- Voltage Sensor2/LConn1 -- Capacitor/RConn1
  Capacitor/LConn1 -- Voltage Sensor2/RConn2 -- Current Sensor1/RConn2
  single_phase_transformer/RConn1 -- Capacitor1/LConn1
  ucs/LConn1 -- Voltage Sensor2/RConn1

== system sst_cllc_dcx_35kHz/dcdc_cllc_modA/dc//dc with galvanic isolation/full-bridge 1 ==
  gate_commands : Inport
  full-full_bridge_ssc_mosfet_based : Subsystem
  uac_1(+) : PMIOPort  Side=Left
  uac_1(-) : PMIOPort  Port=2  Side=Left
  Udc(+) : PMIOPort  Port=3  Side=Right
  Udc(-) : PMIOPort  Port=4  Side=Right
  wires:
  gate_commands/1 -> full-full_bridge_ssc_mosfet_based/1(gate_commands)
  connections:
  full-full_bridge_ssc_mosfet_based/LConn1 -- Udc(+)/RConn1
  full-full_bridge_ssc_mosfet_based/RConn1 -- uac_1(+)/RConn1
  full-full_bridge_ssc_mosfet_based/LConn2 -- Udc(-)/RConn1
  full-full_bridge_ssc_mosfet_based/RConn2 -- uac_1(-)/RConn1

== system sst_cllc_dcx_35kHz/dcdc_cllc_modA/dc//dc with galvanic isolation/full-bridge 2 ==
  gate_commands : Inport
  full_bridge_ssc_mosfet_based : Subsystem
  uac_1(+) : PMIOPort  Side=Left
  uac_1(-) : PMIOPort  Port=2  Side=Left
  Udc(+) : PMIOPort  Port=3  Side=Right
  Udc(-) : PMIOPort  Port=4  Side=Right
  wires:
  gate_commands/1 -> full_bridge_ssc_mosfet_based/1(gate_commands)
  connections:
  full_bridge_ssc_mosfet_based/LConn1 -- Udc(+)/RConn1
  full_bridge_ssc_mosfet_based/RConn1 -- uac_1(+)/RConn1
  full_bridge_ssc_mosfet_based/LConn2 -- Udc(-)/RConn1
  full_bridge_ssc_mosfet_based/RConn2 -- uac_1(-)/RConn1

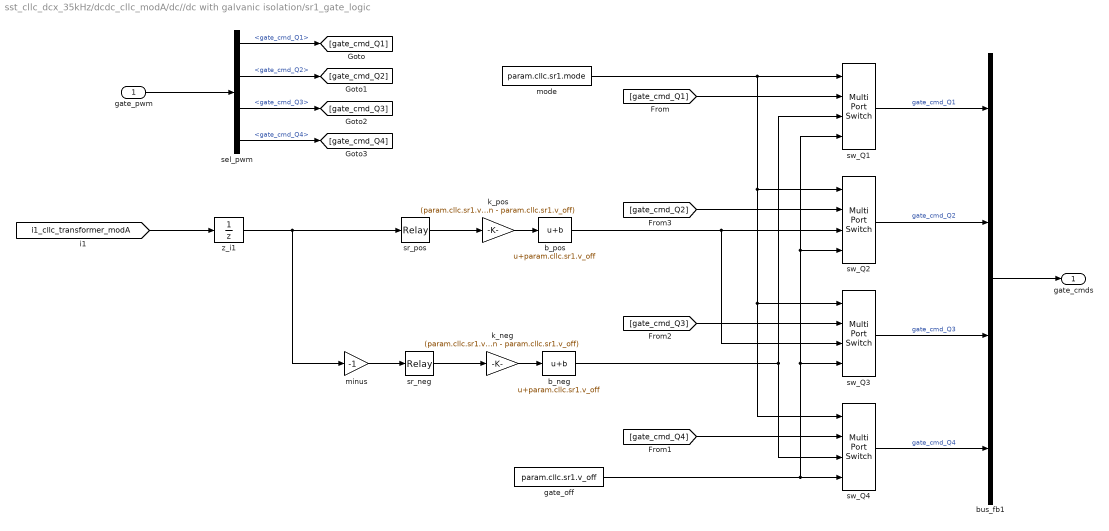
== system sst_cllc_dcx_35kHz/dcdc_cllc_modA/dc//dc with galvanic isolation/sr1_gate_logic ==
  gate_pwm : Inport
  b_neg : Bias  Bias=param.cllc.sr1.v_off  SaturateOnIntegerOverflow=off
  b_pos : Bias  Bias=param.cllc.sr1.v_off  SaturateOnIntegerOverflow=off
  bus_fb1 : BusCreator  Inputs=4
  gate_off : Constant  Value=param.cllc.sr1.v_off
  k_neg : Gain  Gain=(param.cllc.sr1.v_on - param.cllc.sr1.v_off)
  k_pos : Gain  Gain=(param.cllc.sr1.v_on - param.cllc.sr1.v_off)
  minus : Gain  Gain=-1
  mode : Constant  Value=param.cllc.sr1.mode
  sel_pwm : BusSelector  OutputSignals=gate_cmd_Q1,gate_cmd_Q2,gate_cmd_Q3,gate_cmd_Q4
  sr_neg : Relay  OnSwitchValue=param.cllc.sr1.i_on  OffSwitchValue=param.cllc.sr1.i_off
  sr_pos : Relay  OnSwitchValue=param.cllc.sr1.i_on  OffSwitchValue=param.cllc.sr1.i_off
  sw_Q{1..4} (4 alike) : MultiPortSwitch  DataPortOrder=Zero-based contiguous  zeroidx=on  SaturateOnIntegerOverflow=off  InputSameDT=off
  z_i1 : UnitDelay  SampleTime=param.glb_time.tc
  gate_cmds : Outport
  wires:
  gate_pwm/1 -> sel_pwm/1
  [i1_cllc_transformer_modA] -> z_i1/1
  z_i1/1 -> sr_pos/1, minus/1
  minus/1 -> sr_neg/1
  sr_pos/1 -> k_pos/1
  k_pos/1 -> b_pos/1
  sr_neg/1 -> k_neg/1
  k_neg/1 -> b_neg/1
  mode/1 -> sw_Q1/1, sw_Q2/1, sw_Q4/1, sw_Q3/1
  b_neg/1 -> sw_Q4/3, sw_Q1/3
  gate_off/1 -> sw_Q3/4, sw_Q1/4, sw_Q2/4, sw_Q4/4
  sw_Q1/1 -> bus_fb1/1  "gate_cmd_Q1"
  b_pos/1 -> sw_Q3/3, sw_Q2/3
  sw_Q2/1 -> bus_fb1/2  "gate_cmd_Q2"
  sw_Q3/1 -> bus_fb1/3  "gate_cmd_Q3"
  sw_Q4/1 -> bus_fb1/4  "gate_cmd_Q4"
  bus_fb1/1 -> gate_cmds/1
  sel_pwm/1 -> [gate_cmd_Q1]  "<gate_cmd_Q1>"
  sel_pwm/2 -> [gate_cmd_Q2]  "<gate_cmd_Q2>"
  sel_pwm/3 -> [gate_cmd_Q3]  "<gate_cmd_Q3>"
  sel_pwm/4 -> [gate_cmd_Q4]  "<gate_cmd_Q4>"
  [gate_cmd_Q1] -> sw_Q1/2
  [gate_cmd_Q2] -> sw_Q2/2
  [gate_cmd_Q3] -> sw_Q3/2
  [gate_cmd_Q4] -> sw_Q4/2

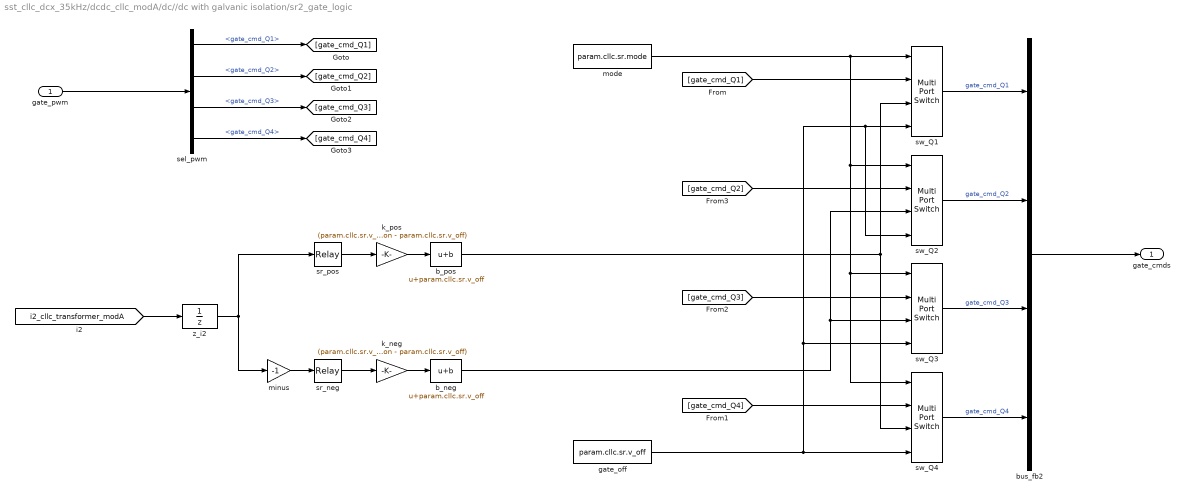
== system sst_cllc_dcx_35kHz/dcdc_cllc_modA/dc//dc with galvanic isolation/sr2_gate_logic ==
  gate_pwm : Inport
  b_neg : Bias  Bias=param.cllc.sr.v_off  SaturateOnIntegerOverflow=off
  b_pos : Bias  Bias=param.cllc.sr.v_off  SaturateOnIntegerOverflow=off
  bus_fb2 : BusCreator  Inputs=4
  gate_off : Constant  Value=param.cllc.sr.v_off
  k_neg : Gain  Gain=(param.cllc.sr.v_on - param.cllc.sr.v_off)
  k_pos : Gain  Gain=(param.cllc.sr.v_on - param.cllc.sr.v_off)
  minus : Gain  Gain=-1
  mode : Constant  Value=param.cllc.sr.mode
  sel_pwm : BusSelector  OutputSignals=gate_cmd_Q1,gate_cmd_Q2,gate_cmd_Q3,gate_cmd_Q4
  sr_neg : Relay  OnSwitchValue=param.cllc.sr.i_on  OffSwitchValue=param.cllc.sr.i_off
  sr_pos : Relay  OnSwitchValue=param.cllc.sr.i_on  OffSwitchValue=param.cllc.sr.i_off
  sw_Q{1..4} (4 alike) : MultiPortSwitch  DataPortOrder=Zero-based contiguous  zeroidx=on  SaturateOnIntegerOverflow=off  InputSameDT=off
  z_i2 : UnitDelay  SampleTime=param.glb_time.tc
  gate_cmds : Outport
  wires:
  gate_pwm/1 -> sel_pwm/1
  [i2_cllc_transformer_modA] -> z_i2/1
  z_i2/1 -> sr_pos/1, minus/1
  minus/1 -> sr_neg/1
  sr_pos/1 -> k_pos/1
  k_pos/1 -> b_pos/1
  sr_neg/1 -> k_neg/1
  k_neg/1 -> b_neg/1
  mode/1 -> sw_Q1/1, sw_Q2/1, sw_Q3/1, sw_Q4/1
  [gate_cmd_Q1] -> sw_Q1/2
  b_pos/1 -> sw_Q4/3, sw_Q1/3
  gate_off/1 -> sw_Q3/4, sw_Q1/4, sw_Q2/4, sw_Q4/4
  sw_Q1/1 -> bus_fb2/1  "gate_cmd_Q1"
  [gate_cmd_Q2] -> sw_Q2/2
  b_neg/1 -> sw_Q3/3, sw_Q2/3
  sw_Q2/1 -> bus_fb2/2  "gate_cmd_Q2"
  [gate_cmd_Q3] -> sw_Q3/2
  sw_Q3/1 -> bus_fb2/3  "gate_cmd_Q3"
  [gate_cmd_Q4] -> sw_Q4/2
  sw_Q4/1 -> bus_fb2/4  "gate_cmd_Q4"
  bus_fb2/1 -> gate_cmds/1
  sel_pwm/1 -> [gate_cmd_Q1]  "<gate_cmd_Q1>"
  sel_pwm/2 -> [gate_cmd_Q2]  "<gate_cmd_Q2>"
  sel_pwm/3 -> [gate_cmd_Q3]  "<gate_cmd_Q3>"
  sel_pwm/4 -> [gate_cmd_Q4]  "<gate_cmd_Q4>"
